simulink model "heat25830_staliro_02"  (Simulink 7.6)
settings: Solver=ode45  StartTime=0.0  StopTime=50  RelTol=1e-5  AbsTol=1e-5
values from neighbouring files (symbols this model uses):
  Amat = [0 0.12 0.08 0 0 0 0 0 0 0.08 0.12 0 ... (100 elements, 10x10)]    [heat30.mat]
  bvec = [0.08 0.1 0.18 0.14 0.14 0.18 0.14 0.18 0.14 0.08]    [heat30.mat]
  cvec = [7 6 5 6 6 5 7 6 6 8]    [heat30.mat]
  dif = [1.5 1.5 0.5 0.5 1.5 1.5 0.5 0.5 1.5 1.5]    [heat30.mat]
  get = [16 17 17 16 15 16 17 16 16 17]    [heat30.mat]
  h = [0 0 1 1 1 0 0 1 0 0]    [heat30.mat]
  rooms = 10    [heat30.mat]
  xinit = [18 18 18 17 18 17 17 17 18 18]    [heat30.mat]
settings Model: Creator=gfaineko  LastModifiedBy=Georgios
settings DataIOCC: LimitDataPoints=off  SaveOutput=off  SignalLogging=off  DSMLogging=off  SaveTime=off  SignalLoggingName=sigsOut
settings DebuggingCC: SaveWithParameterizedLinksMsg=none  SignalResolutionControl=TryResolveAllWithWarning  SolverPrmCheckMsg=none  MultiTaskDSMMsg=warning  MultiTaskCondExecSysMsg=none  InitInArrayFormatMsg=none
settings HardwareCC: TargetUnknown=on
settings SFSimCC: SimParseCustomCode=off
settings RTWCC: IncludeERTFirstTime=on

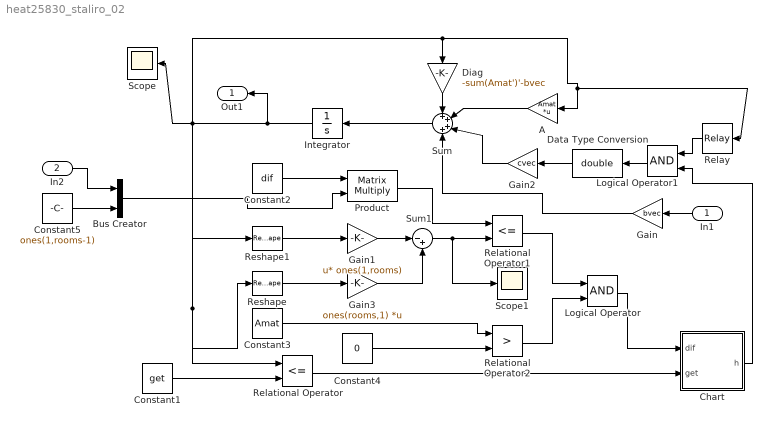
== system heat25830_staliro_02 ==
  In1 : Inport
  In2 : Inport  Port=2
  A : Gain  Gain=Amat  Multiplication=Matrix(K*u)  SaturateOnIntegerOverflow=on  OutDataTypeStr=Inherit: Same as input  ParamDataTypeStr=Inherit: Same as input
  Bus Creator : BusCreator  Inputs=2
  Chart : Stateflow chart  TreatAsAtomicUnit=on
  Constant1 : Constant  Value=get
  Constant2 : Constant  Value=dif
  Constant3 : Constant  Value=Amat  VectorParams1D=off
  Constant4 : Constant  Value=0
  Constant5 : Constant  Value=ones(1,rooms-1)  VectorParams1D=off
  Data Type Conversion : DataTypeConversion  OutDataTypeStr=double  SaturateOnIntegerOverflow=on  RndMeth=Zero
  Diag : Gain  Gain=-sum(Amat')'-bvec  SaturateOnIntegerOverflow=on  OutDataTypeStr=Inherit: Same as input  ParamDataTypeStr=Inherit: Same as input
  Gain : Gain  Gain=bvec  SaturateOnIntegerOverflow=on  OutDataTypeStr=Inherit: Same as input  ParamDataTypeStr=Inherit: Same as input
  Gain1 : Gain  Gain=ones(1,rooms)  Multiplication=Matrix(u*K)  SaturateOnIntegerOverflow=on  OutDataTypeStr=Inherit: Same as input  ParamDataTypeStr=Inherit: Same as input
  Gain2 : Gain  Gain=cvec  SaturateOnIntegerOverflow=on  OutDataTypeStr=Inherit: Same as input  ParamDataTypeStr=Inherit: Same as input
  Gain3 : Gain  Gain=ones(rooms,1)  Multiplication=Matrix(K*u)  SaturateOnIntegerOverflow=on  OutDataTypeStr=Inherit: Same as input  ParamDataTypeStr=Inherit: Same as input
  Integrator : Integrator  InitialCondition=xinit
  Logical Operator : Logic  AllPortsSameDT=off
  Logical Operator1 : Logic  AllPortsSameDT=off
  Product : Product  Multiplication=Matrix(*)  RndMeth=Zero
  Relational Operator : RelationalOperator  Operator=<=  OutDataTypeStr=boolean
  Relational Operator1 : RelationalOperator  Operator=<=  OutDataTypeStr=boolean
  Relational Operator2 : RelationalOperator  Operator=>  OutDataTypeStr=boolean
  Relay : Relay  OnSwitchValue=off  OffSwitchValue=on  OnOutputValue=0  OffOutputValue=1
  Reshape : Reshape  OutputDimensionality=Row vector (2-D)
  Reshape1 : Reshape  OutputDimensionality=Column vector (2-D)
  Scope : Scope
      settings: YMin=15.5  YMax=21.5
  Scope1 : Scope
      settings: YMin=-7.5  YMax=7.5
  Sum : Sum  Inputs=++++  SaturateOnIntegerOverflow=on
  Sum1 : Sum  Inputs=|-+  SaturateOnIntegerOverflow=on
  Out1 : Outport
  wires:
  Sum/1 -> Integrator/1
  Integrator/1 -> Scope/1, Relational Operator/1, Reshape/1, Reshape1/1, Diag/1, Relay/1, A/1, Out1/1
  Diag/1 -> Sum/1
  Relay/1 -> Logical Operator1/1
  Gain/1 -> Sum/4
  In1/1 -> Gain/1
  Relational Operator/1 -> Chart/2(get)
  Constant1/1 -> Relational Operator/2
  Reshape1/1 -> Gain1/1
  Reshape/1 -> Gain3/1
  Gain1/1 -> Sum1/1
  Gain3/1 -> Sum1/2
  Sum1/1 -> Scope1/1, Relational Operator1/2
  Product/1 -> Relational Operator1/1
  Relational Operator1/1 -> Logical Operator/1
  Constant3/1 -> Relational Operator2/1
  Constant4/1 -> Relational Operator2/2
  Relational Operator2/1 -> Logical Operator/2
  Logical Operator/1 -> Chart/1(dif)
  Logical Operator1/1 -> Data Type Conversion/1
  Data Type Conversion/1 -> Gain2/1
  Chart/1(h) -> Logical Operator1/2
  A/1 -> Sum/2
  Gain2/1 -> Sum/3
  Constant5/1 -> Bus Creator/2
  In2/1 -> Bus Creator/1
  Constant2/1 -> Product/1
  Bus Creator/1 -> Product/2

== stateflow chart Chart ==
  state main [parallel]
    settings: executionOrder=1
    main -> (junction 4) : {id1=0;id2=0;}
    (junction 4) -> (junction 9) [order 1] : [id1<rooms]
    (junction 11) -> (junction 6) [order 1] : [id2<rooms]
    (junction 6) -> (junction 7)
    (junction 13) -> (junction 11)
    (junction 9) -> (junction 16)
    (junction 8) -> (junction 4)
    (junction 14) -> (junction 8) : {id1++;}
    (junction 16) -> (junction 11) [order 1] : [get[id1]&!h[id1]]
    (junction 11) -> (junction 5) [order 2] : {id2=0;}
    (junction 12) -> (junction 10)
    (junction 7) -> (junction 13) [order 2] : {id2++;}
    (junction 10) -> main
    (junction 15) -> (junction 12) : {h[id1]=1;h[id2]=0;}
    (junction 7) -> (junction 15) [order 1] : [dif[id1][id2]&h[id2]]
    (junction 5) -> (junction 14)
    (junction 16) -> (junction 14) [order 2]
    (junction 4) -> (junction 10) [order 2]
  data: id1 local int16; id2 local int16; rooms parameter double; dif input boolean size=10,10; get input boolean size=10; h output double size=10
